simulink model "test2_tempconv"  (R2025b)
settings: Solver=VariableStepAuto  StartTime=0.0  StopTime=10.0  RelTol=1e-3
values from neighbouring files (symbols this model uses):
  X = input(prompt)    [project2.m]
settings Model: Creator=Shriram  LastModifiedBy=Shriram

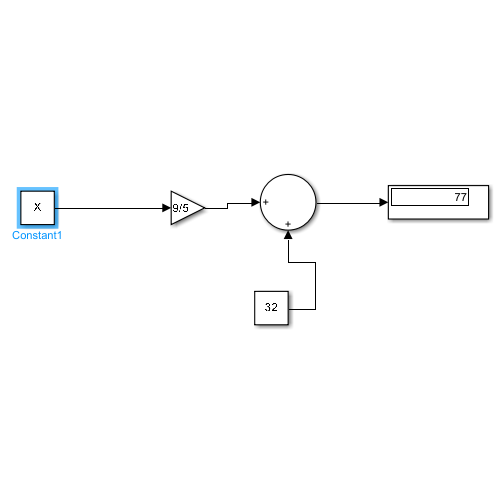
[thumbnail: Simulink's stored preview of the top-level diagram]
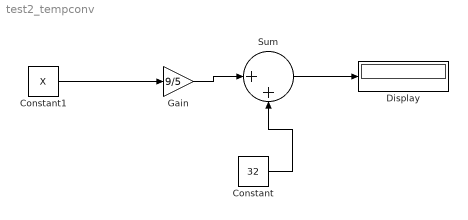
== system test2_tempconv ==
  Constant : Constant  Value=32
  Constant1 : Constant  Value=X
  Display : Display
  Gain : Gain  Gain=9/5
  Sum : Sum  Inputs=|++
  wires:
  Constant/1 -> Sum/2
  Gain/1 -> Sum/1
  Sum/1 -> Display/1
  Constant1/1 -> Gain/1
